simulink model "ZF02HD250606_23a"  (R2023a)
settings: Solver=ode4  StartTime=0.0  StopTime=inf  FixedStep=0.002  RelTol=1e-3
InitFcn:
  |  T_c = 0.002;
undefined symbols (not defined in the file): DiscIntNeverNeededParam, Discrete, magnitude, Time
libraries: AFCToolbox x33, simulink x28, simulink_extras x7, sharedtransform x2, ctrlSharedLib x2, aerolibconvert2 x1, aerolibtransform2 x1, dspstat3 x1, dspsolvers x1
(part 1 of 3)
settings Model: Creator=zqinghua  LastModifiedBy=zqhkd
settings OptimizationCC: DefaultParameterBehavior=Inlined  OptimizeBlockIOStorage=off  BufferReuse=off  ReuseModelBlockBuffer=off  GlobalBufferReuse=off  ExpressionFolding=off  EnableMemcpy=off  PassReuseOutputArgsAs=Individual arguments  LocalBlockOutputs=off  ZeroExternalMemoryAtStartup=off  ZeroInternalMemoryAtStartup=off  OptimizeDataStoreBuffers=off  BusAssignmentInplaceUpdate=off  OptimizationLevel=level0  OptimizationCustomize=off  EfficientTunableParamExpr=on
settings DebuggingCC: ParameterOverflowMsg=none  ParameterUnderflowMsg=error  ParameterTunabilityLossMsg=error
settings HardwareCC: ProdBitPerInt=16  ProdBitPerPointer=16  ProdBitPerSizeT=16  ProdBitPerPtrDiffT=16  ProdLargestAtomicFloat=None  ProdWordSize=16  ProdHWDeviceType=STMicroelectronics->ST10/Super10  TargetBitPerInt=16  TargetBitPerPointer=16  TargetBitPerSizeT=16  TargetBitPerPtrDiffT=16  TargetIntDivRoundTo=Zero  TargetEndianess=LittleEndian  TargetWordSize=16  TargetHWDeviceType=STMicroelectronics->ST10/Super10
settings SFSimCC: MATLABDynamicMemAlloc=off
settings RTWCC: Description=Embedded Coder  SystemTargetFile=AFCHawk.tlc  GenCodeOnly=on  TemplateMakefile=ert_default_tmf
settings CodeAppCC: ForceParamTrailComments=on  IgnoreCustomStorageClasses=off  OperatorAnnotations=on  SimulinkDataObjDesc=on  SFDataObjDesc=on  InsertBlockDesc=on
settings STFCustomTargetCC: MultiwordLength=256  ModelReferenceCompliant=off  ConcurrentExecutionCompliant=off  CombineOutputUpdateFcns=on  ERTCustomFileBanners=on  SupportContinuousTime=off  SupportNonInlinedSFcns=off  RemoveResetFunc=on  MATLABClassNameForMDSCustomization=Simulink.SoftwareTarget.ERTCustomization  GRTInterface=off  UseToolchainInfoCompliant=off  SystemTargetFile=AFCHawk.tlc
settings ERTTargetCC: TargetLangStandard=C99 (ISO)  ModelReferenceCompliant=off  ParMdlRefBuildCompliant=off  CompOptLevelCompliant=off  ConcurrentExecutionCompliant=off  ModelStepFunctionPrototypeControlCompliant=off  CPPClassGenCompliant=off  UseToolchainInfoCompliant=off  InlinedParameterPlacement=NonHierarchical  ERTCustomFileTemplate=example_file_process.tlc
settings ConfigComp: CovBoundaryAbsTol=1.0e-5

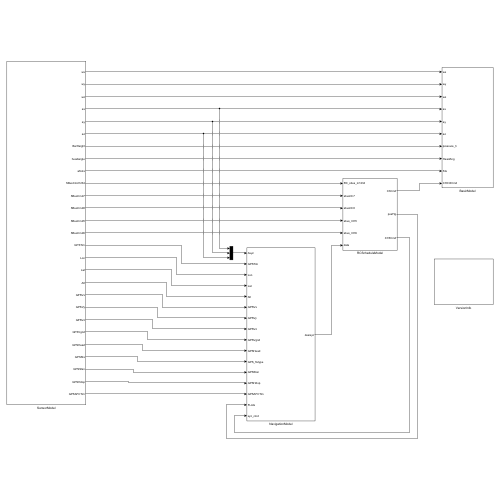
[thumbnail: Simulink's stored preview of the top-level diagram]
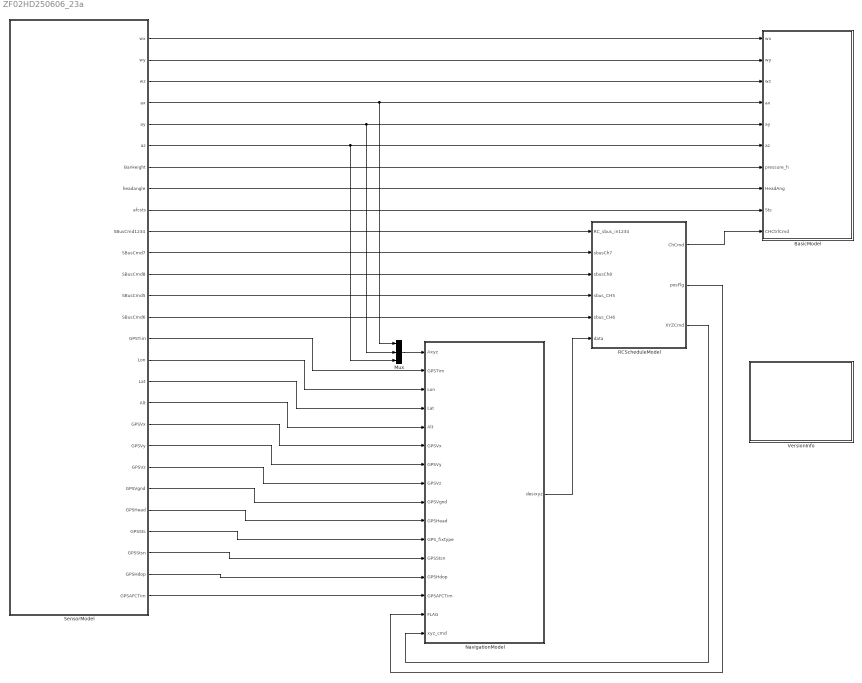
== system ZF02HD250606_23a ==
  BasicModel : Subsystem
  Mux : Mux  Inputs=3
  NavigationModel : Subsystem
  RCScheduleModel : Subsystem
  SensorModel : Subsystem
  VersionInfo : Subsystem
  wires:
  RCScheduleModel/1(ChCmd) -> BasicModel/10(CHCtrlCmd)
  SensorModel/8(headangle) -> BasicModel/8(HeadAng)
  SensorModel/21(GPSVz) -> NavigationModel/8(GPSVz)
  SensorModel/20(GPSVy) -> NavigationModel/7(GPSVy)
  SensorModel/23(GPSHead) -> NavigationModel/10(GPSHead)
  SensorModel/4(ax) -> Mux/1, BasicModel/4(ax)
  SensorModel/18(Alt) -> NavigationModel/5(Alt)
  SensorModel/25(GPSStsn) -> NavigationModel/12(GPSStsn)
  SensorModel/17(Lat) -> NavigationModel/4(Lat)
  SensorModel/19(GPSVx) -> NavigationModel/6(GPSVx)
  SensorModel/7(BarHeight) -> BasicModel/7(pressure_h)
  RCScheduleModel/3(XYZCmd) -> NavigationModel/16(xyz_cmd)
  NavigationModel/1(desixyz) -> RCScheduleModel/6(data)
  SensorModel/27(GPSAFCTim) -> NavigationModel/14(GPSAFCTim)
  SensorModel/16(Lon) -> NavigationModel/3(Lon)
  SensorModel/24(GPSSts) -> NavigationModel/11(GPS_fixtype)
  RCScheduleModel/2(posFlg) -> NavigationModel/15(FLAG)
  SensorModel/9(afcsts) -> BasicModel/9(Sts)
  SensorModel/15(GPSTim) -> NavigationModel/2(GPSTim)
  SensorModel/1(wx) -> BasicModel/1(wx)
  SensorModel/26(GPSHdop) -> NavigationModel/13(GPSHdop)
  SensorModel/12(SBusCmd8) -> RCScheduleModel/3(sbusCh8)
  SensorModel/11(SBusCmd7) -> RCScheduleModel/2(sbusCh7)
  SensorModel/14(SBusCmd6) -> RCScheduleModel/5(sbus_CH6)
  SensorModel/22(GPSVgnd) -> NavigationModel/9(GPSVgnd)
  SensorModel/10(SBusCmd1234) -> RCScheduleModel/1(RC_sbus_in1234)
  SensorModel/6(az) -> Mux/3, BasicModel/6(az)
  SensorModel/3(wz) -> BasicModel/3(wz)
  SensorModel/13(SBusCmd5) -> RCScheduleModel/4(sbus_CH5)
  SensorModel/2(wy) -> BasicModel/2(wy)
  SensorModel/5(ay) -> Mux/2, BasicModel/5(ay)
  Mux/1 -> NavigationModel/1(Axyz)

== system ZF02HD250606_23a/BasicModel ==
  note: 起飞前检查数据
  note: 飞行分析用的详细监测数据
  wx : Inport
  wy : Inport  Port=2
  wz : Inport  Port=3
  ax : Inport  Port=4
  ay : Inport  Port=5
  az : Inport  Port=6
  pressure_h : Inport  Port=7
  HeadAng : Inport  Port=8
  Sts : Inport  Port=9
  CHCtrlCmd : Inport  Port=10
  AttiAltHold : Subsystem
  Data Type Conversion : DataTypeConversion  OutDataTypeStr=double  SaturateOnIntegerOverflow=off  RndMeth=Floor
  Tx02 : Subsystem
  Tx03 : Subsystem
  ZF02无人机 : Subsystem  Priority=6
  tag scope: flySts=global, pwm=global
  wires:
  pressure_h/1 -> AttiAltHold/7(pressure_h)
  wz/1 -> AttiAltHold/3(Wz)
  wy/1 -> AttiAltHold/2(Wy)
  wx/1 -> AttiAltHold/1(Wx)
  ax/1 -> AttiAltHold/4(Ax)
  az/1 -> AttiAltHold/6(Az)
  ay/1 -> AttiAltHold/5(Ay)
  CHCtrlCmd/1 -> AttiAltHold/10(CHCtrlCmd)
  HeadAng/1 -> AttiAltHold/8(HeadAng)
  Sts/1 -> AttiAltHold/9(Sts)
  AttiAltHold/1(MotorOut) -> ZF02无人机/1(MotorVal), [pwm]
  AttiAltHold/2(flySts) -> ZF02无人机/2(FlySts), Data Type Conversion/1
  Data Type Conversion/1 -> [flySts]

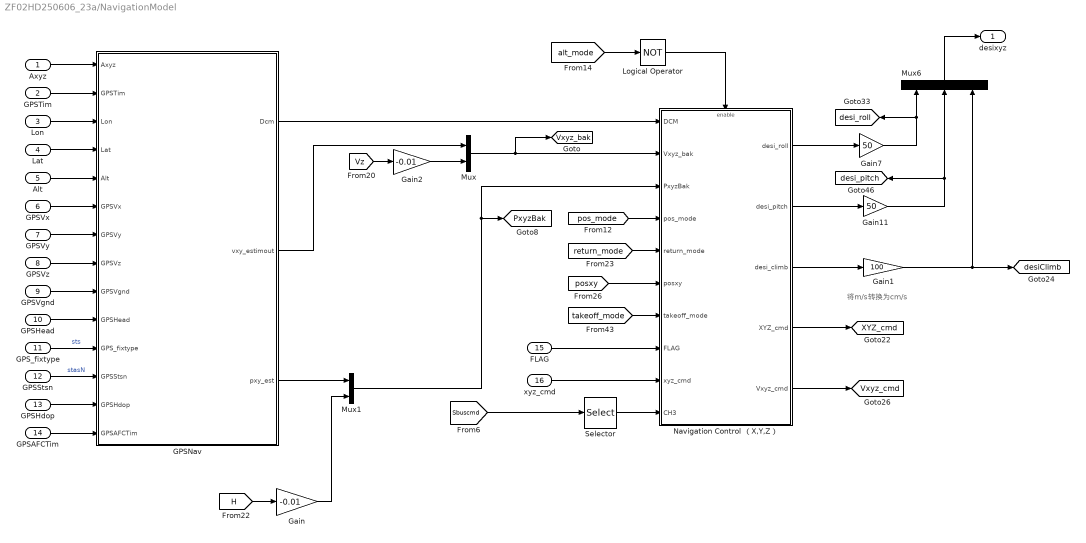
== system ZF02HD250606_23a/NavigationModel ==
  note: 将m/s转换为cm/s
  Axyz : Inport
  GPSTim : Inport  Port=2
  Lon : Inport  Port=3
  Lat : Inport  Port=4
  Alt : Inport  Port=5
  GPSVx : Inport  Port=6
  GPSVy : Inport  Port=7
  GPSVz : Inport  Port=8
  GPSVgnd : Inport  Port=9
  GPSHead : Inport  Port=10
  GPS_fixtype : Inport  Port=11
  GPSStsn : Inport  Port=12
  GPSHdop : Inport  Port=13
  GPSAFCTim : Inport  Port=14
  FLAG : Inport  Port=15
  xyz_cmd : Inport  Port=16
  " Navigation Control （X,Y,Z）" : Subsystem
  GPSNav : Subsystem
  Gain : Gain  Gain=-0.01
  Gain1 : Gain  Gain=100
  Gain11 : Gain  Gain=50
  Gain2 : Gain  Gain=-0.01
  Gain7 : Gain  Gain=50
  Logical Operator : Logic  Operator=NOT  AllPortsSameDT=off  OutDataTypeStr=boolean
  Mux : Mux  Inputs=2
  Mux1 : Mux  Inputs=2
  Mux6 : Mux  Inputs=3
  Selector : Selector  InputPortWidth=4  IndexOptions=Index vector (dialog)  Indices=3  OutputSizes=1
  desixyz : Outport
  tag scope: PxyzBak=global, Vxyz_bak=global, Vxyz_cmd=global, XYZ_cmd=global, desiClimb=global, desi_pitch=global, desi_roll=global
  wires:
  xyz_cmd/1 -> " Navigation Control （X,Y,Z）"/9(xyz_cmd)
  Mux6/1 -> desixyz/1
  FLAG/1 -> " Navigation Control （X,Y,Z）"/8(FLAG)
  Gain1/1 -> Mux6/3, [desiClimb]
  [H] -> Gain/1
  [takeoff_mode] -> " Navigation Control （X,Y,Z）"/7(takeoff_mode)
  " Navigation Control （X,Y,Z）"/3(desi_climb) -> Gain1/1
  [pos_mode] -> " Navigation Control （X,Y,Z）"/4(pos_mode)
  Logical Operator/1 -> " Navigation Control （X,Y,Z）"/Enable
  [return_mode] -> " Navigation Control （X,Y,Z）"/5(return_mode)
  [posxy] -> " Navigation Control （X,Y,Z）"/6(posxy)
  " Navigation Control （X,Y,Z）"/1(desi_roll) -> Gain7/1
  " Navigation Control （X,Y,Z）"/2(desi_pitch) -> Gain11/1
  " Navigation Control （X,Y,Z）"/4(XYZ_cmd) -> [XYZ_cmd]
  " Navigation Control （X,Y,Z）"/5(Vxyz_cmd) -> [Vxyz_cmd]
  Gain7/1 -> Mux6/1, [desi_roll]
  Gain11/1 -> Mux6/2, [desi_pitch]
  GPSTim/1 -> GPSNav/2(GPSTim)
  Lon/1 -> GPSNav/3(Lon)
  Lat/1 -> GPSNav/4(Lat)
  Alt/1 -> GPSNav/5(Alt)
  GPSVx/1 -> GPSNav/6(GPSVx)
  GPSVy/1 -> GPSNav/7(GPSVy)
  GPSVz/1 -> GPSNav/8(GPSVz)
  GPSVgnd/1 -> GPSNav/9(GPSVgnd)
  GPSHead/1 -> GPSNav/10(GPSHead)
  GPS_fixtype/1 -> GPSNav/11(GPS_fixtype)  "sts"
  GPSStsn/1 -> GPSNav/12(GPSStsn)  "stasN"
  GPSHdop/1 -> GPSNav/13(GPSHdop)
  GPSAFCTim/1 -> GPSNav/14(GPSAFCTim)
  [alt_mode] -> Logical Operator/1
  GPSNav/1(Dcm) -> " Navigation Control （X,Y,Z）"/1(DCM)
  GPSNav/2(vxy_estimout) -> Mux/1
  Axyz/1 -> GPSNav/1(Axyz)
  [Sbuscmd] -> Selector/1
  Selector/1 -> " Navigation Control （X,Y,Z）"/10(CH3)
  Mux/1 -> [Vxyz_bak], " Navigation Control （X,Y,Z）"/2(Vxyz_bak)
  [Vz] -> Gain2/1
  Gain2/1 -> Mux/2
  GPSNav/3(pxy_est) -> Mux1/1
  Gain/1 -> Mux1/2
  Mux1/1 -> " Navigation Control （X,Y,Z）"/3(PxyzBak), [PxyzBak]

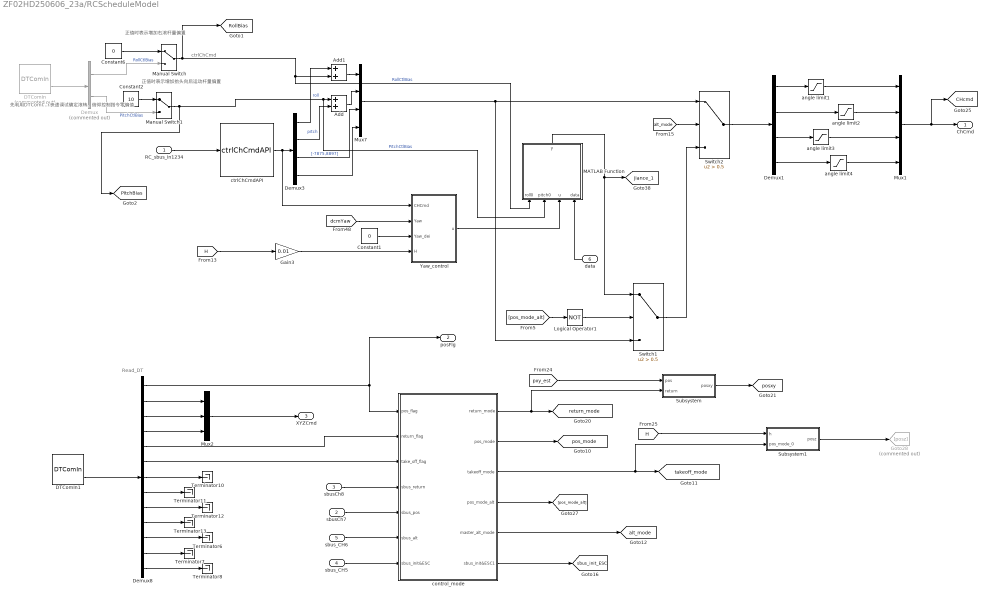
== system ZF02HD250606_23a/RCScheduleModel ==
  note: 先利用DTComIn快速调试确定滚转、俯仰控制指令零偏值
  note: 正值时表示增加右滚杆量偏置
  note: ctrlChCmd
  note: Read_DT
  note: 正值时表示增加抬头向后运动杆量偏置
  RC_sbus_in1234 : Inport
  sbusCh7 : Inport  Port=2
  sbusCh8 : Inport  Port=3
  sbus_CH5 : Inport  Port=4
  sbus_CH6 : Inport  Port=5
  data : Inport  Port=6
  Add : Sum
  Add1 : Sum
  Constant1 : Constant  Value=0
  Constant2 : Constant  Value=10
  Constant6 : Constant  Value=0
  DTComIn : AFCToolbox/DeviceModule/DTComIn  Priority=2  Commented=on  g_sampleTime=0.01  g_frameType=22  g_resFrameNum=0  g_comPort=6  g_instName=0  g_id=0
      settings: SourceProductName=AFCToolbox
  DTComIn1 : AFCToolbox/DeviceModule/DTComIn  Priority=2  g_sampleTime=0.01  g_frameType=25  g_resFrameNum=0  g_comPort=6  g_instName=0  g_id=0
      settings: SourceProductName=AFCToolbox
  Demux : Demux  Commented=on  Outputs=2
  Demux1 : Demux
  Demux3 : Demux
  Demux8 : Demux  Outputs=13
  Gain3 : Gain  Gain=0.01
  Goto28 : Goto  Commented=on  GotoTag=posz
  Logical Operator1 : Logic  Operator=NOT  AllPortsSameDT=off  OutDataTypeStr=boolean
  MATLAB Function : MATLAB Function  TreatAsAtomicUnit=on
  Manual Switch : ManualSwitch
  Manual Switch1 : ManualSwitch
  Mux1 : Mux
  Mux2 : Mux  Inputs=3
  Mux7 : Mux
  Subsystem : Subsystem
  Subsystem1 : Subsystem
  Switch1 : Switch  Criteria=u2 > Threshold  Threshold=0.5  SaturateOnIntegerOverflow=off  InputSameDT=off
  Switch2 : Switch  Criteria=u2 > Threshold  Threshold=0.5  SaturateOnIntegerOverflow=off  InputSameDT=off
  Terminator{6..8,10..13} (7 alike) : Terminator
  Yaw_control : Subsystem
  angle limit1 : Saturate  UpperLimit=1500  LowerLimit=-1500
  angle limit2 : Saturate  UpperLimit=1500  LowerLimit=-1500
  angle limit3 : Saturate  UpperLimit=10500  LowerLimit=-10500
  angle limit4 : Saturate  UpperLimit=250  LowerLimit=-250
  control_mode : Subsystem
  ctrlChCmdAPI : AFCToolbox/APPModule/ctrlChCmdAPI  Priority=3
      settings: SourceProductName=AFCToolbox
  ChCmd : Outport
  posFlg : Outport  Port=2
  XYZCmd : Outport  Port=3
  tag scope: CHcmd=global, PitchBias=global, RollBias=global, alt_mode=global, jiance_1=global, pos_mode=global, posxy=global, return_mode=global, sbus_init_ESC=global, takeoff_mode=global
  wires:
  Demux3/4 -> Mux7/4
  [pxy_est] -> Subsystem/1(pos)
  [pos_mode_alt] -> Logical Operator1/1
  ctrlChCmdAPI/1 -> Demux3/1, Yaw_control/1(CHCmd)
  Switch1/1 -> Switch2/3
  Manual Switch/1 -> [RollBias], Add1/2, MATLAB Function/1(roll0)  "RollCtlBias"
  Manual Switch1/1 -> [PitchBias], MATLAB Function/2(pitch0), Add/1  "PitchCtlBias"
  Add1/1 -> Mux7/1
  Demux3/1 -> Add1/1  "roll"
  Demux8/11 -> Terminator6/1
  Demux8/1 -> posFlg/1, control_mode/1(pos_flag)
  Demux3/2 -> Add/2  "pitch"
  Demux3/3 -> Mux7/3  "[-7875,8897]"
  Add/1 -> Mux7/2
  Mux7/1 -> Switch1/3, Switch2/1
  Demux8/3 -> Mux2/2
  Demux8/2 -> Mux2/1
  Demux8/4 -> Mux2/3
  [alt_mode] -> Switch2/2
  Demux8/7 -> Terminator10/1
  [H] -> Subsystem1/1(h)
  Demux8/8 -> Terminator11/1
  Demux8/9 -> Terminator12/1
  sbusCh8/1 -> control_mode/4(sbus_return)
  Demux8/10 -> Terminator13/1
  Yaw_control/1(u) -> MATLAB Function/3(u)
  Demux8/12 -> Terminator7/1
  Demux8/13 -> Terminator8/1
  control_mode/4(pos_mode_alt) -> [pos_mode_alt]
  RC_sbus_in1234/1 -> ctrlChCmdAPI/1
  control_mode/3(takeoff_mode) -> [takeoff_mode], Subsystem1/2(pos_mode_0)
  [H] -> Gain3/1
  sbusCh7/1 -> control_mode/5(sbus_pos)
  [dcmYaw] -> Yaw_control/2(Yaw)
  Constant1/1 -> Yaw_control/3(Yaw_dei)
  Gain3/1 -> Yaw_control/4(H)
  sbus_CH6/1 -> control_mode/6(sbus_alt)
  sbus_CH5/1 -> control_mode/7(sbus_init&ESC)
  control_mode/1(return_mode) -> Subsystem/2(return), [return_mode]
  control_mode/2(pos_mode) -> [pos_mode]
  control_mode/5(master_alt_mode) -> [alt_mode]
  control_mode/6(sbus_init&ESC1) -> [sbus_init_ESC]
  MATLAB Function/1(y) -> Switch1/1, [jiance_1]
  Logical Operator1/1 -> Switch1/2
  Subsystem1/1(posz) -> Goto28/1
  Subsystem/1(posxy) -> [posxy]
  data/1 -> MATLAB Function/4(data)
  Demux8/6 -> control_mode/3(take_off_flag)
  Demux8/5 -> control_mode/2(return_flag)
  Mux2/1 -> XYZCmd/1
  DTComIn1/2 -> Demux8/1
  angle limit3/1 -> Mux1/3
  angle limit4/1 -> Mux1/4
  Demux1/4 -> angle limit4/1
  angle limit1/1 -> Mux1/1
  Switch2/1 -> Demux1/1
  angle limit2/1 -> Mux1/2
  Demux1/2 -> angle limit2/1
  Mux1/1 -> [CHcmd], ChCmd/1
  Demux1/3 -> angle limit3/1
  Demux1/1 -> angle limit1/1
  DTComIn/2 -> Demux/1
  Demux/1 -> Manual Switch/2  "RollCtlBias"
  Constant6/1 -> Manual Switch/1
  Demux/2 -> Manual Switch1/2  "PitchCtlBias"
  Constant2/1 -> Manual Switch1/1

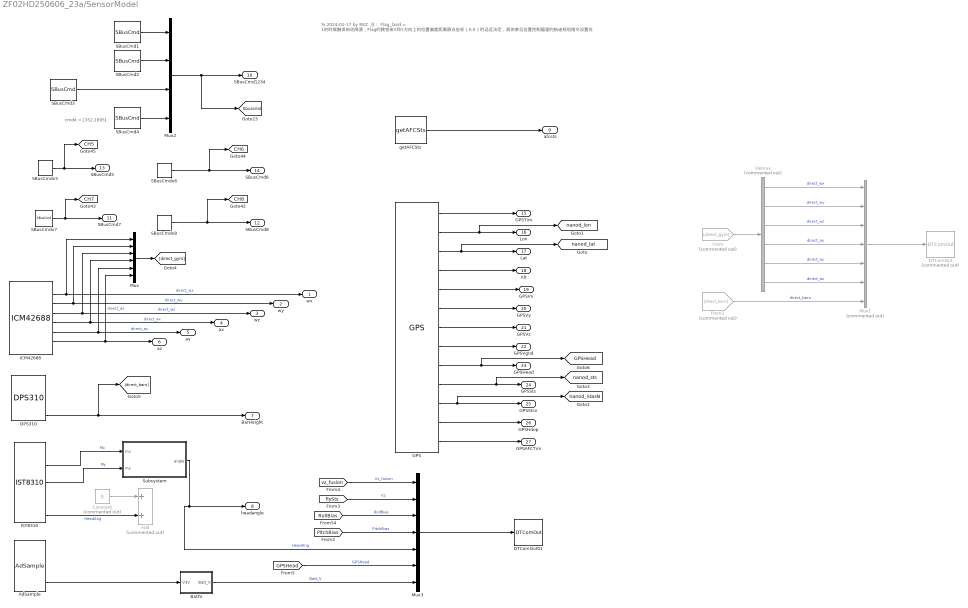
== system ZF02HD250606_23a/SensorModel ==
  note: % 2024-01-17 by REZ
      | 注：
      | Flag_land = 1的时候触发自动降落，Flag的跳变由X和Y方向上的位置偏差距离原点坐标（0,0）的远近决定，具体参见位置控制器里的航迹规划指令设置处
  note: cmd4 = [352,1695]
  AdSample : AFCToolbox/DeviceModule/AdSample  Priority=1  g_sampleTime=0.01  g_comPort=0  g_instName=0  g_id=0
      settings: SourceProductName=AFCToolbox
  Add : Sum  Commented=on
  BattV : Subsystem
  Constant : Constant  Commented=on  Value=0
  DPS310 : AFCToolbox/DeviceModule/DPS310  Priority=1  g_sampleTime=0.01  g_comPort=6  g_instName=0  g_id=0
      settings: SourceProductName=AFCToolbox
  DTComOut : AFCToolbox/DeviceModule/DTComOut  Priority=8  Commented=on  g_frameType=4  g_outFreq=10  g_comPort=0  g_instName=0  g_id=0
      settings: SourceProductName=AFCToolbox
  DTComOut01 : AFCToolbox/DeviceModule/DTComOut  Priority=8  g_frameType=1  g_outFreq=30  g_comPort=0  g_instName=0  g_id=0
      settings: SourceProductName=AFCToolbox
  Demux : Demux  Commented=on  Outputs=6
  From : From  Commented=on  GotoTag=direct_gyro
  From1 : From  Commented=on  GotoTag=direct_baro
  GPS : AFCToolbox/DeviceModule/GPS  Priority=1  g_sampleTime=T_c  g_gpsDev=M10 GNSS  g_comPort=6  g_instName=0  g_id=0
      settings: SourceProductName=AFCToolbox
  ICM42688 : AFCToolbox/DeviceModule/ICM42688  Priority=0  g_sampleTime=T_c  g_comPort=6  g_instName=0  g_id=0
      settings: SourceProductName=AFCToolbox
  IST8310 : AFCToolbox/DeviceModule/IST8310  Priority=1  g_sampleTime=0.01  g_comPort=0  g_instName=0  g_id=0
      settings: SourceProductName=AFCToolbox
  Mux : Mux  Inputs=6
  Mux1 : Mux  Commented=on  Inputs=7
  Mux2 : Mux
  Mux3 : Mux  Inputs=7
  SBusCmd1 : AFCToolbox/DeviceModule/SBusCmd  Priority=0  g_sampleTime=T_c  g_chanelNo=1  g_comPort=6  g_instName=0  g_id=0
      settings: SourceProductName=AFCToolbox
  SBusCmd2 : AFCToolbox/DeviceModule/SBusCmd  Priority=0  g_sampleTime=T_c  g_chanelNo=2  g_comPort=6  g_instName=0  g_id=0
      settings: SourceProductName=AFCToolbox
  SBusCmd3 : AFCToolbox/DeviceModule/SBusCmd  Priority=0  g_sampleTime=T_c  g_chanelNo=3  g_comPort=6  g_instName=0  g_id=0
      settings: SourceProductName=AFCToolbox
  SBusCmd4 : AFCToolbox/DeviceModule/SBusCmd  Priority=0  g_sampleTime=T_c  g_chanelNo=4  g_comPort=6  g_instName=0  g_id=0
      settings: SourceProductName=AFCToolbox
  SBusCmdx5 : AFCToolbox/DeviceModule/SBusCmd  Priority=0  g_sampleTime=T_c  g_chanelNo=5  g_comPort=6  g_instName=0  g_id=0
      settings: SourceProductName=AFCToolbox
  SBusCmdx6 : AFCToolbox/DeviceModule/SBusCmd  Priority=0  g_sampleTime=T_c  g_chanelNo=6  g_comPort=6  g_instName=0  g_id=0
      settings: SourceProductName=AFCToolbox
  SBusCmdx7 : AFCToolbox/DeviceModule/SBusCmd  Priority=0  g_sampleTime=0.002  g_chanelNo=7  g_comPort=6  g_instName=0  g_id=0
      settings: SourceProductName=AFCToolbox
  SBusCmdx8 : AFCToolbox/DeviceModule/SBusCmd  Priority=0  g_sampleTime=T_c  g_chanelNo=8  g_comPort=6  g_instName=0  g_id=0
      settings: SourceProductName=AFCToolbox
  Subsystem : Subsystem
  getAFCSts : AFCToolbox/APPModule/getAFCSts  Priority=0  g_sampleTime=T_c
      settings: SourceProductName=AFCToolbox
  wx : Outport
  wy : Outport  Port=2
  wz : Outport  Port=3
  ax : Outport  Port=4
  ay : Outport  Port=5
  az : Outport  Port=6
  BarHeight : Outport  Port=7
  headangle : Outport  Port=8
  afcsts : Outport  Port=9
  SBusCmd1234 : Outport  Port=10
  SBusCmd7 : Outport  Port=11
  SBusCmd8 : Outport  Port=12
  SBusCmd5 : Outport  Port=13
  SBusCmd6 : Outport  Port=14
  GPSTim : Outport  Port=15
  Lon : Outport  Port=16
  Lat : Outport  Port=17
  Alt : Outport  Port=18
  GPSVx : Outport  Port=19
  GPSVy : Outport  Port=20
  GPSVz : Outport  Port=21
  GPSVgnd : Outport  Port=22
  GPSHead : Outport  Port=23
  GPSSts : Outport  Port=24
  GPSStsn : Outport  Port=25
  GPSHdop : Outport  Port=26
  GPSAFCTim : Outport  Port=27
  tag scope: CH5=global, CH6=global, CH7=global, CH8=global, GPSHead=global, Sbuscmd=global, nanod_StasN=global, nanod_lat=global, nanod_lon=global, nanod_sts=global
  wires:
  GPS/1 -> GPSTim/1
  GPS/2 -> [nanod_lon], Lon/1
  GPS/3 -> [nanod_lat], Lat/1
  GPS/4 -> Alt/1
  SBusCmd1/1 -> Mux2/1
  SBusCmd2/1 -> Mux2/2
  SBusCmd3/1 -> Mux2/3
  SBusCmd4/1 -> Mux2/4
  SBusCmdx7/1 -> [CH7], SBusCmd7/1
  getAFCSts/1 -> afcsts/1
  SBusCmdx8/1 -> [CH8], SBusCmd8/1
  SBusCmdx6/1 -> [CH6], SBusCmd6/1
  GPS/12 -> GPSHdop/1
  DPS310/4 -> [direct_baro], BarHeight/1
  GPS/11 -> GPSStsn/1, [nanod_StasN]
  ICM42688/2 -> Mux/1, wx/1  "direct_wx"
  ICM42688/5 -> Mux/4, ax/1  "direct_ax"
  GPS/7 -> GPSVz/1
  GPS/8 -> GPSVgnd/1
  SBusCmdx5/1 -> [CH5], SBusCmd5/1
  GPS/5 -> GPSVx/1
  GPS/6 -> GPSVy/1
  GPS/9 -> [GPSHead], GPSHead/1
  GPS/10 -> [nanod_sts], GPSSts/1
  GPS/13 -> GPSAFCTim/1
  Mux2/1 -> [Sbuscmd], SBusCmd1234/1
  ICM42688/3 -> Mux/2, wy/1  "direct_wy"
  ICM42688/6 -> Mux/5, ay/1  "direct_ay"
  ICM42688/4 -> Mux/3, wz/1  "direct_wz"
  ICM42688/7 -> Mux/6, az/1  "direct_az"
  Mux/1 -> [direct_gyro]
  From1/1 -> Mux1/7  "direct_baro"
  Demux/6 -> Mux1/6  "direct_az"
  Mux1/1 -> DTComOut/1
  Demux/1 -> Mux1/1  "direct_wx"
  Demux/2 -> Mux1/2  "direct_wy"
  Demux/4 -> Mux1/4  "direct_ax"
  Demux/3 -> Mux1/3  "direct_wz"
  Demux/5 -> Mux1/5  "direct_ay"
  From/1 -> Demux/1
  Subsystem/1(angle) -> Mux3/5, headangle/1  "HeadAng"
  AdSample/3 -> BattV/1(V3V)
  Mux3/1 -> DTComOut01/1
  [RollBias] -> Mux3/3  "RollBias"
  [flySts] -> Mux3/2  "Vz"
  [vz_fusion] -> Mux3/1  "Vz_fusion"
  [PitchBias] -> Mux3/4  "PitchBias"
  BattV/1(Batt_V) -> Mux3/7  "Batt_V"
  IST8310/5 -> Add/2  "HeadAng"
  Constant/1 -> Add/1
  [GPSHead] -> Mux3/6  "GPSHead"
  IST8310/3 -> Subsystem/2(my)  "My"
  IST8310/2 -> Subsystem/1(mx)  "Mx"

== system ZF02HD250606_23a/VersionInfo ==
  note: % 2024-01-11 Positon Controller 修改 ， by REZ
      |
      | 1.积分器重置条件，根据油门，已知实际遥控器CH3>0.4左右开始离地，离地前需要进行积分器重置； 遥控器的CH3=0.3-0.4左右对应在模型中Cmd_ch3=880，即重置条件为：当Ch3<880进行积分重置。
      |
      | 2.积分器的限幅范围：对位置控制器里的四个积分器暂时施加了[-3,3]的限幅，主要考虑当x和y方向的位置误差最大在3m内的时候，单纯由积分器得到的控制量不能占据PID控制器主导量而导致控制异常！
      |
      | %2024-01-15:
      | 位置控制器重修，P-PID控制器参数修改了一版；积分限幅
      |
      | % 2024-01-16：
      | 修改增加了一个含逻辑切换的正方形航迹规划指令；
      |
      | %2024-01-19:
      | 航迹规划的优化及飞行验证；
      |
      | %22024-03-08：
      | 增加control_mode模式选择模块：
      | （1）ch5为sbus_init_ESC开关同时进行电调控制解锁与导航初始化，其不受其他模式影响；
      | （2）ch6为高度控制与位置模式的切换通道，通道置1为高度控制模式，否则将进行位置控制模式，在所有模式中高度控制模式优先级最高，只要该通道置1，其他模式将不起作用；
      | （3）ch7为位置控制模式，该模式优先级最低，主要进行航迹飞行，其他通道置零，ch7通道置1，进行预设点飞行，否则进入（0,0,h）定点模式，定点模式可以理解为航迹规划前的无人机位置调整与准备；
      | （4）ch8为返航控制模式，该模式优先级高于航迹控制，但低于高度控制模式，通道置1，无人机将进行返航任务。
      |
      | %22024-03-08：
      | 优化位置控制模块，可随意更改航迹点，并预留与上位机进行点位设置的接口模块。注意，该版本航迹飞行为平面飞行，未涉及到高度，因此在进行点位设置时，只需设计X和Y两个方向的点位，可自行在setpoints封装模块的MASK界面进行修改，同时可修改触发阈值。
      |
      | %22024-03-10：
      | 优化位置控制，同时增加返航模块。将位置控制模式划分为三个模 式，（0,0）定点模式，航迹规划模式，一键返航模式，与control_mode相对应，通过遥控器对应拨杆进行模式切换。
      | （1）三个模式共用同一组控制参数，（0,0）定点模式和航迹规划模式不进行高度控制，保持当前高度；
      | （2）一键返航模式任务要求，无人机接收到指令后，首先保持水平位置，进行高度方向的飞行，达到决断高度之后，无人机保持当前高度h0,然后向（0,0,h）点位飞行，随后无人机进行降落。
      | （3）将位置模式产生的上升率与下降率叠加到遥控器指令生成的控制率中。
      |
      | %22024-03-11：
      | 优化位置控制，可进行三维空间点位设置。
      |
      | %22024-03-12：
      | 取消pos_mode(0,0)模式，优化三维航迹，无人机接受指令后，先飞行高度，随后进行水平飞行。
      |
      | %22024-03-14：
      | 优化返航模式，解决了返航复飞的现象。
      |
      | %22024-03-14：
      | 增加了定点模式，航迹飞行前，无人机先进行当前高度的单定点飞行，验证其飞行性能，随后进行三维航迹飞行。
      |
      | %22024-03-14：
      | 加入偏航控制模式，使其一直处于正北方向。
      |
      | %22024-03-15：
      | 增加上位机点位设置模块。
      |
      | %22024-03-16：
      | 将偏航控制单独加到位置控制模式；
      |
      | %22024-03-17：
      | 增加一键起飞模式，无人机解锁，同时油门至中位，此时，将遥控器7号拨杆至中位，无人机进行一键起飞。
      |
      | %22024-03-18：
      | 简化三维航迹飞行，同时进行高度与水平飞行。
      | %22024-03-22：
      | 优化偏航控制，在飞行高度大于0.5米，偏航控制有效。
      | %22024-03-24：
      | 优化上位机控制逻辑，实现遥控控制与上位机控制相互兼容，上位机可发送起飞指令，返航指令，三维坐标点。
      | %22024-05-15:
      | F550-4 飞8m；未加磁力计补偿，yaw的kp参数需要在线调参为6.6；
      |
      | %22024-11-05:
      | HS03 飞行正常；
      |
      | %2024-11-09：
      | . 删除SensorModel中的DTComIn, 将相应功能移至RCScheduleModel模块中；
      | . 恢复HS620PN241105.slx中setpoints1、return_mode1中删除的微分跟踪器TD模块；
      | . 在control_mode模块中，对于位置、起飞/降落等模块的触发设置一个总开关与模块PosCtlSwitch，以防止T20241105_111134出现的故障；
      |
      | V5.05.241204：根据HS620PN241111(T20241112_083920飞行的V2.424版本更改)

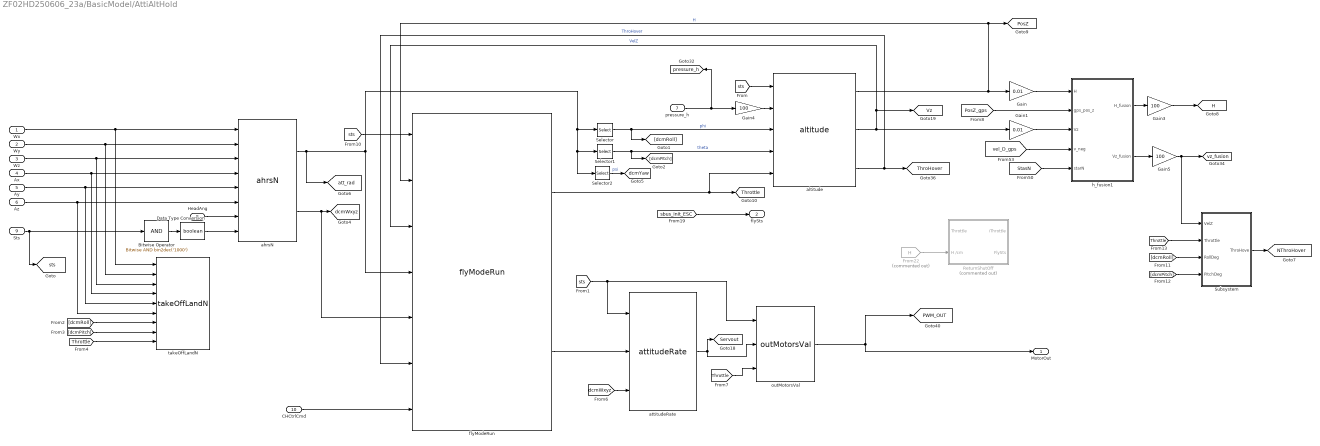
== system ZF02HD250606_23a/BasicModel/AttiAltHold ==
  Wx : Inport
  Wy : Inport  Port=2
  Wz : Inport  Port=3
  Ax : Inport  Port=4
  Ay : Inport  Port=5
  Az : Inport  Port=6
  pressure_h : Inport  Port=7
  HeadAng : Inport  Port=8
  Sts : Inport  Port=9
  CHCtrlCmd : Inport  Port=10
  Bitwise Operator : simulink/Logic and Bit Operations/Bitwise Operator  logicop=AND  UseBitMask=on  BitMask=bin2dec('1000')  BitMaskRealWorld=Stored Integer
  Data Type Conversion : DataTypeConversion  OutDataTypeStr=boolean  SaturateOnIntegerOverflow=off  RndMeth=Floor
  From22 : From  Commented=on  GotoTag=H  TagVisibility=global
  Gain : Gain  Gain=0.01
  Gain1 : Gain  Gain=0.01
  Gain3 : Gain  Gain=100
  Gain4 : Gain  Gain=100
  Gain5 : Gain  Gain=100
  ReturnShutOff : Subsystem  Commented=on
  Selector : Selector  InputPortWidth=3  IndexOptions=Index vector (dialog)  Indices=1  OutputSizes=1
  Selector1 : Selector  InputPortWidth=3  IndexOptions=Index vector (dialog)  Indices=2  OutputSizes=1
  Selector2 : Selector  InputPortWidth=3  IndexOptions=Index vector (dialog)  Indices=3  OutputSizes=1
  Subsystem : Subsystem
  ahrsN : AFCToolbox/APPModule/ahrsN  Priority=3  kp=0.14  ki=0.0087  kp_yaw=0.16  ki_yaw=0.001  dt=0.002  g=9.80665
      settings: SourceProductName=AFCToolbox
  altitude : AFCToolbox/APPModule/altitude  Priority=3  alt_pos_kp=1.8  pid_alt_rate_kp=8.0  pid_alt_rate_ki=0.1  pid_alt_rate_kd=1.0  pid_alt_rate_imax=800.0  pid_alt_accel_kp=1.36  pid_alt_accel_ki=0.1  pid_alt_accel_kd=0.08  pid_alt_accel_imax=800.0  k1=0.6  k2=0.12  k3=0.008  control_dt=0.002  g=9.80665
      settings: SourceProductName=AFCToolbox
  attitudeRate : AFCToolbox/APPModule/attitudeRate  Priority=4  angle_kp0=8.0  angle_kp1=6.6  angle_kp2=8.0  pid_rate0_kp=0.32  pid_rate0_ki=0.1  pid_rate0_kd=3.5  pid_rate1_kp=0.32  pid_rate1_ki=0.1  pid_rate1_kd=3.5  pid_rate2_kp=0.6  pid_rate2_ki=0.03  pid_rate2_kd=1.5  pid_rate0_imax=500.0  pid_rate1_imax=500.0  pid_rate2_imax=500.0  max0=5000.0  min0=-5000.0  max1=5000.0  min1=-5000.0  max2=4000.0  min2=-4000.0  control_dt=0.002
      settings: SourceProductName=AFCToolbox
  flyModeRun : AFCToolbox/APPModule/flyModeRun  Priority=4
      settings: SourceProductName=AFCToolbox
  h_fusion1 : Subsystem
  outMotorsVal : AFCToolbox/APPModule/outMotorsVal  Priority=5
      settings: SourceProductName=AFCToolbox
  takeOffLandN : AFCToolbox/APPModule/takeOffLandN  Priority=5  RC_Climb_Rate=0
      settings: SourceProductName=AFCToolbox
  MotorOut : Outport
  flySts : Outport  Port=2
  tag scope: H=global, NThroHover=global, PWM_OUT=global, PosZ=global, Servout=global, ThroHover=global, Throttle=global, Vz=global, att_rad=global, dcmWxyz=global, dcmYaw=global, pressure_h=global, sts=global, vz_fusion=global
  wires:
  Selector1/1 -> [dcmPitch], altitude/4  "theta"
  Data Type Conversion/1 -> ahrsN/8
  ahrsN/2 -> flyModeRun/5, [dcmWxyz]
  attitudeRate/1 -> outMotorsVal/2, [Servout]
  Selector/1 -> altitude/3, [dcmRoll]  "phi"
  Ax/1 -> takeOffLandN/4, ahrsN/4
  Wx/1 -> takeOffLandN/1, ahrsN/1
  [Throttle] -> takeOffLandN/9
  ahrsN/1 -> [att_rad], flyModeRun/4, Selector2/1, Selector1/1, Selector/1
  [dcmRoll] -> takeOffLandN/7
  [dcmPitch] -> takeOffLandN/8
  [sts] -> altitude/1
  [dcmWxyz] -> attitudeRate/3
  outMotorsVal/1 -> MotorOut/1, [PWM_OUT]
  Selector2/1 -> [dcmYaw]  "psi"
  flyModeRun/2 -> attitudeRate/2
  [Throttle] -> outMotorsVal/3
  [sts] -> attitudeRate/1, outMotorsVal/1
  altitude/3 -> [ThroHover], flyModeRun/6  "ThroHover"
  [sts] -> flyModeRun/1
  Gain4/1 -> altitude/2
  pressure_h/1 -> [pressure_h], Gain4/1
  CHCtrlCmd/1 -> flyModeRun/7
  HeadAng/1 -> ahrsN/7
  Sts/1 -> [sts], Bitwise Operator/1
  Bitwise Operator/1 -> Data Type Conversion/1
  Wy/1 -> takeOffLandN/2, ahrsN/2
  Wz/1 -> takeOffLandN/3, ahrsN/3
  Ay/1 -> takeOffLandN/5, ahrsN/5
  Az/1 -> takeOffLandN/6, ahrsN/6
  altitude/2 -> Gain1/1, [Vz], flyModeRun/3  "VelZ"
  altitude/1 -> [PosZ], flyModeRun/2, Gain/1  "H"
  [dcmRoll] -> Subsystem/3(RollDeg)
  [dcmPitch] -> Subsystem/4(PitchDeg)
  Gain5/1 -> Subsystem/1(VelZ), [vz_fusion]
  Subsystem/1(ThroHove) -> [NThroHover]
  [Throttle] -> Subsystem/2(Throttle)
  [PosZ_gps] -> h_fusion1/2(gps_pos_z)
  h_fusion1/1(H_fusion) -> Gain3/1
  Gain/1 -> h_fusion1/1(H)
  Gain3/1 -> [H]
  Gain1/1 -> h_fusion1/3(Vz)
  [vel_D_gps] -> h_fusion1/4(v_neg)
  [StasN] -> h_fusion1/5(starN)
  h_fusion1/2(Vz_fusion) -> Gain5/1
  [sbus_init_ESC] -> flySts/1
  From22/1 -> ReturnShutOff/2(H /cm)
  flyModeRun/1 -> altitude/5, [Throttle]

== system ZF02HD250606_23a/BasicModel/Tx02 ==
  DTComOut2 : AFCToolbox/DeviceModule/DTComOut  Priority=8  g_frameType=2  g_outFreq=10  g_comPort=0  g_instName=0  g_id=0
      settings: SourceProductName=AFCToolbox
  Demux1 : Demux
  Demux12 : Demux
  Demux6 : Demux  Outputs=3
  Mux : Mux  Inputs=26
  Radians to Degrees2 : simulink_extras/Transformations/Radians to Degrees
  Subsystem2 : Subsystem
  wires:
  [pos_N_gps] -> Mux/1  "pos_N_gps"
  Demux12/2 -> Mux/16  "CH2"
  Demux6/1 -> Mux/12  "att_deg_roll"
  [CH6] -> Mux/21  "CH6"
  [nanod_sts] -> Mux/5  "nanod_sts"
  [PosZ_gps] -> Mux/3  "PosZ_gps"
  [pos_E_gps] -> Mux/2  "pos_E_gps"
  [att_rad] -> Radians to Degrees2/1
  [CH8] -> Mux/19  "CH8"
  [Sbuscmd] -> Demux12/1
  [nanod_lon] -> Mux/9, Subsystem2/2(lon_in)  "nanod_lon"
  [pressure_h] -> Mux/4  "pressure_h"
  [nanod_lat] -> Subsystem2/1(lat_in), Mux/8  "nanod_lat"
  Subsystem2/2(lon_out) -> Mux/11  "lon_jieduan"
  Radians to Degrees2/1 -> Demux6/1
  [CH5] -> Mux/22  "CH5"
  [nanod_StasN] -> Mux/7  "nanod_StasN"
  Subsystem2/1(lat_out) -> Mux/10  "lat_jieduan"
  [CH7] -> Mux/20  "CH7"
  Demux12/3 -> Mux/17  "CH3"
  Demux6/2 -> Mux/13  "att_deg_pitch"
  Demux12/4 -> Mux/18  "CH4"
  Demux6/3 -> Mux/14  "att_deg_yaw"
  Demux12/1 -> Mux/15  "CH1"
  Mux/1 -> DTComOut2/1
  Demux1/4 -> Mux/26  "CHCmd4"
  Demux1/3 -> Mux/25  "CHCmd3"
  Demux1/2 -> Mux/24  "CHCmd2"
  Demux1/1 -> Mux/23  "CHCmd1"
  [CHcmd] -> Demux1/1
  [PosZ] -> Mux/6  "PosZ"

== system ZF02HD250606_23a/BasicModel/Tx03 ==
  DTComOut2 : AFCToolbox/DeviceModule/DTComOut  Priority=8  g_frameType=3  g_outFreq=10  g_comPort=0  g_instName=0  g_id=0
      settings: SourceProductName=AFCToolbox
  Data Type Conversion : DataTypeConversion  OutDataTypeStr=double  SaturateOnIntegerOverflow=off  RndMeth=Floor
  Demux{,1,3..4,6} (5 alike) : Demux  Outputs=3
  Demux2 : Demux
  Mux : Mux  Inputs=26
  wires:
  [dcmWxyz] -> Demux4/1
  Demux/3 -> Mux/7  "pz_bak"
  Demux/1 -> Mux/5  "px_bak"
  Demux/2 -> Mux/6  "py_bak"
  Demux1/3 -> Mux/13  "vz_bak"
  Demux1/1 -> Mux/11  "vx_bak"
  Demux1/2 -> Mux/12  "vy_bak"
  Demux4/1 -> Mux/14  "dcmWx"
  Demux4/2 -> Mux/15  "dcmWy"
  Demux4/3 -> Mux/16  "dcmWz"
  Mux/1 -> DTComOut2/1
  [PxyzBak] -> Demux/1
  [Vxyz_bak] -> Demux1/1
  [pwm] -> Demux2/1
  Demux2/4 -> Mux/4  "pwm4"
  Demux2/3 -> Mux/3  "pwm3"
  Demux2/2 -> Mux/2  "pwm2"
  Demux2/1 -> Mux/1  "pwm1"
  Demux3/1 -> Mux/8  "vx_cmd"
  Demux3/2 -> Mux/9  "vy_cmd"
  Demux3/3 -> Mux/10  "vz_cmd"
  [Vxyz_cmd] -> Demux3/1
  [Throttle] -> Mux/20  "Throttle"
  Data Type Conversion/1 -> Mux/21  "AFC5Sts"
  [sts] -> Data Type Conversion/1
  [desi_roll] -> Mux/22  "desiRoll"
  [desi_pitch] -> Mux/23  "desiPitch"
  [desiClimb] -> Mux/24  "desiH"
  [ThroHover] -> Mux/25  "HoverThrottle"
  [H] -> Mux/26  "PosZ_fusion"
  Demux6/1 -> Mux/17  "X_cmd"
  Demux6/2 -> Mux/18  "Y_cmd"
  Demux6/3 -> Mux/19  "Z_cmd"
  [XYZ_cmd] -> Demux6/1  "PitchBias"

== system ZF02HD250606_23a/BasicModel/ZF02无人机 ==
  MotorVal : Inport
  FlySts : Inport  Port=2
  Constant : Constant  Value=0  OutDataTypeStr=double
  Demux1 : Demux
  HiEscCmd : AFCToolbox/DeviceModule/HiEscCmd  Priority=6  g_chanelNo=4  g_minPW=40  g_maxPW=80  g_comPort=6  g_instName=0  g_id=0
      settings: SourceProductName=AFCToolbox
  HiEscCmd1 : AFCToolbox/DeviceModule/HiEscCmd  Priority=6  g_chanelNo=5  g_minPW=40  g_maxPW=80  g_comPort=6  g_instName=0  g_id=0
      settings: SourceProductName=AFCToolbox
  HiEscCmd2 : AFCToolbox/DeviceModule/HiEscCmd  Priority=6  g_chanelNo=6  g_minPW=40  g_maxPW=80  g_comPort=6  g_instName=0  g_id=0
      settings: SourceProductName=AFCToolbox
  HiEscCmd3 : AFCToolbox/DeviceModule/HiEscCmd  Priority=6  g_chanelNo=3  g_minPW=40  g_maxPW=80  g_comPort=6  g_instName=0  g_id=0
      settings: SourceProductName=AFCToolbox
  Mux : Mux
  Switch1 : Switch  Criteria=u2 > Threshold  Threshold=0.5  SaturateOnIntegerOverflow=off  InputSameDT=off
  wires:
  MotorVal/1 -> Switch1/1
  FlySts/1 -> Switch1/2
  Switch1/1 -> Demux1/1
  Mux/1 -> Switch1/3
  Constant/1 -> Mux/4, Mux/3, Mux/2, Mux/1
  Demux1/1 -> HiEscCmd/1  "pwm1"
  Demux1/2 -> HiEscCmd1/1  "pwm2"
  Demux1/3 -> HiEscCmd2/1  "pwm3"
  Demux1/4 -> HiEscCmd3/1  "pwm4"

== system ZF02HD250606_23a/NavigationModel/ Navigation Control （X,Y,Z） ==
  DCM : Inport
  Vxyz_bak : Inport  Port=2
  PxyzBak : Inport  Port=3
  pos_mode : Inport  Port=4
  return_mode : Inport  Port=5
  posxy : Inport  Port=6
  takeoff_mode : Inport  Port=7
  FLAG : Inport  Port=8
  xyz_cmd : Inport  Port=9
  CH3 : Inport  Port=10
  Enable : EnablePort
  Compare To Constant : simulink/Logic and Bit Operations/Compare To Constant  relop=<=  const=800  OutDataTypeStr=boolean
  Logical Operator : Logic  Operator=OR  AllPortsSameDT=off  OutDataTypeStr=boolean
  POS_CONTROL : Subsystem
  SETPOINT : Subsystem
  VEL_PID : Subsystem
  desi_roll : Outport
  desi_pitch : Outport  Port=2
  desi_climb : Outport  Port=3
  XYZ_cmd : Outport  Port=4
  Vxyz_cmd : Outport  Port=5
  wires:
  VEL_PID/1(desi_roll) -> desi_roll/1
  VEL_PID/2(desi_pitch) -> desi_pitch/1
  VEL_PID/3(desi_climb) -> desi_climb/1
  return_mode/1 -> SETPOINT/3(return_mode)
  pos_mode/1 -> SETPOINT/2(pos_mode)
  SETPOINT/1(XYZ_cmd) -> XYZ_cmd/1, POS_CONTROL/1(XYZ_cmd)
  POS_CONTROL/1(Vxyz_cmd) -> Vxyz_cmd/1, VEL_PID/1(Vxyz_cmd)
  DCM/1 -> VEL_PID/2(DCM)
  Vxyz_bak/1 -> VEL_PID/3(Vxyz_bak)
  posxy/1 -> SETPOINT/1(posxy)
  takeoff_mode/1 -> SETPOINT/4(takeoff_mode)
  xyz_cmd/1 -> SETPOINT/5(xyz_cmd)
  FLAG/1 -> SETPOINT/6(FLAG)
  Logical Operator/1 -> VEL_PID/4(ClrKi), POS_CONTROL/3(ClrKi)
  CH3/1 -> Compare To Constant/1
  Compare To Constant/1 -> Logical Operator/2
  SETPOINT/2(Flag) -> Logical Operator/1
  PxyzBak/1 -> POS_CONTROL/2(XYZ_bak), SETPOINT/7(XYZ_bak)

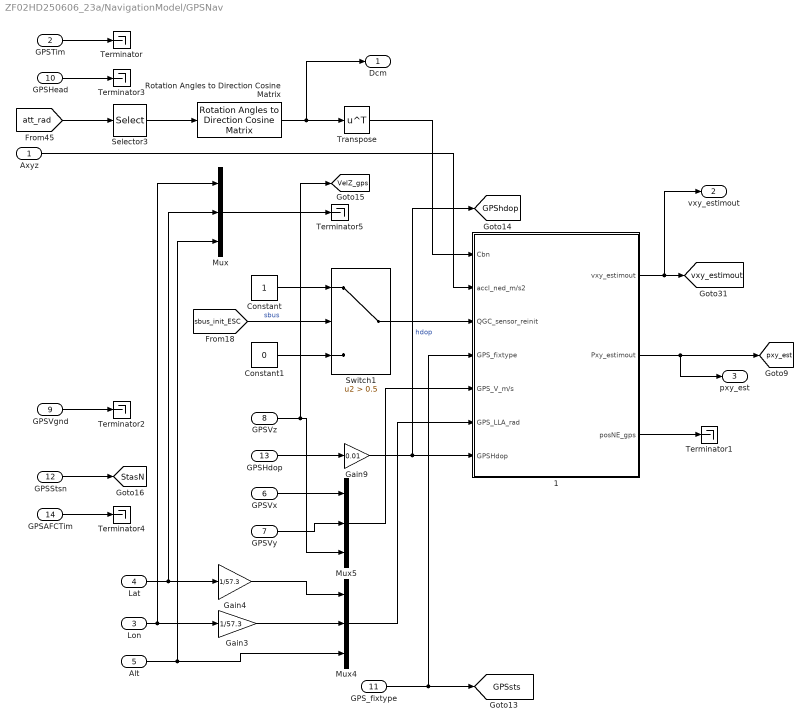
== system ZF02HD250606_23a/NavigationModel/GPSNav ==
  Axyz : Inport
  GPSTim : Inport  Port=2
  Lon : Inport  Port=3
  Lat : Inport  Port=4
  Alt : Inport  Port=5
  GPSVx : Inport  Port=6
  GPSVy : Inport  Port=7
  GPSVz : Inport  Port=8
  GPSVgnd : Inport  Port=9
  GPSHead : Inport  Port=10
  GPS_fixtype : Inport  Port=11
  GPSStsn : Inport  Port=12
  GPSHdop : Inport  Port=13
  GPSAFCTim : Inport  Port=14
  1 : Subsystem  mask{dt=0.002}
      mask prompts: dt "步长"
      mask DialogControl ParameterGroupVar Prompt: 参数
  Constant : Constant
  Constant1 : Constant  Value=0
  Gain3 : Gain  Gain=1/57.3
  Gain4 : Gain  Gain=1/57.3
  Gain9 : Gain  Gain=0.01
  Mux : Mux  Inputs=3
  Mux4 : Mux  Inputs=3
  Mux5 : Mux  Inputs=3
  Rotation Angles to Direction Cosine Matrix : sharedtransform/Rotation Angles to Direction Cosine Matrix  rotationOrder=ZYX  aMode=aMode
  Selector3 : Selector  InputPortWidth=3  IndexOptions=Index vector (dialog)  Indices=[3 2 1]  OutputSizes=1
  Switch1 : Switch  Criteria=u2 > Threshold  Threshold=0.5  SaturateOnIntegerOverflow=off  InputSameDT=off
  Terminator{,1..5} (6 alike) : Terminator
  Transpose : Math  Operator=transpose
  Dcm : Outport
  vxy_estimout : Outport  Port=2
  pxy_est : Outport  Port=3
  tag scope: GPShdop=global, GPSsts=global, StasN=global, VelZ_gps=global, pxy_est=global, vxy_estimout=global
  wires:
  GPSTim/1 -> Terminator/1
  GPSVz/1 -> [VelZ_gps], Mux5/3
  GPSStsn/1 -> [StasN]
  GPSVgnd/1 -> Terminator2/1
  GPSHead/1 -> Terminator3/1
  Gain3/1 -> Mux4/2
  Mux/1 -> Terminator5/1
  [att_rad] -> Selector3/1
  Selector3/1 -> Rotation Angles to Direction Cosine Matrix/1
  Axyz/1 -> 1/2(accl_ned_m/s2)
  GPSAFCTim/1 -> Terminator4/1
  Lat/1 -> Gain4/1, Mux/2
  GPSVy/1 -> Mux5/2
  Lon/1 -> Gain3/1, Mux/1
  Alt/1 -> Mux4/3, Mux/3
  Rotation Angles to Direction Cosine Matrix/1 -> Transpose/1, Dcm/1
  Constant1/1 -> Switch1/3
  [sbus_init_ESC] -> Switch1/2  "sbus"
  Constant/1 -> Switch1/1
  GPSHdop/1 -> Gain9/1
  GPSVx/1 -> Mux5/1
  Gain4/1 -> Mux4/1
  Transpose/1 -> 1/1(Cbn)
  Switch1/1 -> 1/3(QGC_sensor_reinit)
  Mux4/1 -> 1/6(GPS_LLA_rad)
  Gain9/1 -> 1/7(GPSHdop), [GPShdop]  "hdop"
  Mux5/1 -> 1/5(GPS_V_m/s)
  GPS_fixtype/1 -> [GPSsts], 1/4(GPS_fixtype)
  1/1(vxy_estimout) -> [vxy_estimout], vxy_estimout/1
  1/2(Pxy_estimout) -> pxy_est/1, [pxy_est]
  1/3(posNE_gps) -> Terminator1/1

== system ZF02HD250606_23a/RCScheduleModel/Subsystem ==
  pos : Inport
  return : Inport  Port=2
  Logical Operator : Logic  Operator=NOT  AllPortsSameDT=off  OutDataTypeStr=boolean
  Memory : Memory
  Switch : Switch  Criteria=u2 > Threshold  Threshold=0.5  SaturateOnIntegerOverflow=off  InputSameDT=off
  posxy : Outport
  wires:
  Switch/1 -> Memory/1, posxy/1
  Memory/1 -> Switch/3
  return/1 -> Logical Operator/1
  pos/1 -> Switch/1
  Logical Operator/1 -> Switch/2

== system ZF02HD250606_23a/RCScheduleModel/Subsystem1 ==
  h : Inport
  pos_mode_0 : Inport  Port=2
  Gain : Gain  Gain=-0.01
  Logical Operator : Logic  Operator=NOT  AllPortsSameDT=off  OutDataTypeStr=boolean
  Memory : Memory
  Switch : Switch  Criteria=u2 > Threshold  Threshold=0.5  SaturateOnIntegerOverflow=off  InputSameDT=off
  posz : Outport
  wires:
  Logical Operator/1 -> Switch/2
  h/1 -> Gain/1
  pos_mode_0/1 -> Logical Operator/1
  Memory/1 -> Switch/3
  Switch/1 -> posz/1, Memory/1
  Gain/1 -> Switch/1

== system ZF02HD250606_23a/RCScheduleModel/Yaw_control ==
  CHCmd : Inport
  Yaw : Inport  Port=2
  Yaw_dei : Inport  Port=3
  H : Inport  Port=4
  Demux9 : Demux
  MATLAB Function2 : MATLAB Function  TreatAsAtomicUnit=on
  Mux7 : Mux
  Switch : Switch  Criteria=u2 > Threshold  Threshold=0.5  SaturateOnIntegerOverflow=off  InputSameDT=off
  u : Outport
  wires:
  Demux9/1 -> Mux7/1
  Demux9/4 -> Mux7/4
  Demux9/3 -> Switch/3, MATLAB Function2/1(u)  "[-7875,8897]"
  Demux9/2 -> Mux7/2
  Mux7/1 -> u/1
  Yaw/1 -> MATLAB Function2/2(Yaw)
  CHCmd/1 -> Demux9/1
  Yaw_dei/1 -> MATLAB Function2/3(Yaw_dei)
  MATLAB Function2/1(des_wz) -> Switch/1
  H/1 -> Switch/2
  Switch/1 -> Mux7/3

== system ZF02HD250606_23a/RCScheduleModel/control_mode ==
  pos_flag : Inport
  return_flag : Inport  Port=2
  take_off_flag : Inport  Port=3
  sbus_return : Inport  Port=4
  sbus_pos : Inport  Port=5
  sbus_alt : Inport  Port=6
  sbus_init&ESC : Inport  Port=7
  Compare To Constant{,1,3..4} (4 alike) : simulink/Logic and Bit Operations/Compare To Constant  relop=>=  const=1500  OutDataTypeStr=boolean
  Compare To Constant2 : simulink/Logic and Bit Operations/Compare To Constant  relop=<  const=1500  OutDataTypeStr=boolean
  Compare To Constant5 : simulink/Logic and Bit Operations/Compare To Constant  relop=<  const=800  OutDataTypeStr=boolean
  Compare To Constant6 : simulink/Logic and Bit Operations/Compare To Constant  relop=>=  const=800  OutDataTypeStr=boolean
  Compare To Constant7 : simulink/Logic and Bit Operations/Compare To Constant  relop=>=  const=0.5  OutDataTypeStr=boolean
  Compare To Constant8 : simulink/Logic and Bit Operations/Compare To Constant  relop=>=  const=0.5  OutDataTypeStr=boolean
  Compare To Constant9 : simulink/Logic and Bit Operations/Compare To Constant  relop=>=  const=0.5  OutDataTypeStr=boolean
  Logical Operator{,3,10..11} (4 alike) : Logic  Operator=NOT  AllPortsSameDT=off  OutDataTypeStr=boolean
  Logical Operator1 : Logic  Inputs=3  AllPortsSameDT=off  OutDataTypeStr=boolean
  Logical Operator2 : Logic  Inputs=4  AllPortsSameDT=off  OutDataTypeStr=boolean
  Logical Operator4 : Logic  AllPortsSameDT=off  OutDataTypeStr=boolean
  Logical Operator5 : Logic  AllPortsSameDT=off  OutDataTypeStr=boolean
  Logical Operator6 : Logic  Inputs=5  AllPortsSameDT=off  OutDataTypeStr=boolean
  Logical Operator7 : Logic  Operator=OR  AllPortsSameDT=off  OutDataTypeStr=boolean
  Logical Operator8 : Logic  Operator=OR  AllPortsSameDT=off  OutDataTypeStr=boolean
  Logical Operator9 : Logic  Operator=OR  AllPortsSameDT=off  OutDataTypeStr=boolean
  PosCtlSwitch : Logic  AllPortsSameDT=off  OutDataTypeStr=boolean
  return_mode : Outport
  pos_mode : Outport  Port=2
  takeoff_mode : Outport  Port=3
  pos_mode_alt : Outport  Port=4
  master_alt_mode : Outport  Port=5
  sbus_init&ESC1 : Outport  Port=6
  tag scope: CH5_BOOL=global
  wires:
  Logical Operator4/1 -> Logical Operator/1, return_mode/1
  Logical Operator/1 -> Logical Operator6/4, Logical Operator2/3, Logical Operator1/1
  sbus_return/1 -> Compare To Constant/1
  Compare To Constant1/1 -> Logical Operator8/2
  Logical Operator1/1 -> pos_mode/1, Logical Operator11/1
  Compare To Constant2/1 -> Logical Operator5/1
  Logical Operator2/1 -> Logical Operator10/1, takeoff_mode/1
  sbus_alt/1 -> Compare To Constant3/1
  Compare To Constant3/1 -> master_alt_mode/1, Logical Operator3/1
  Compare To Constant/1 -> Logical Operator7/2
  PosCtlSwitch/1 -> Logical Operator4/2, Logical Operator1/3, Logical Operator2/4, Logical Operator6/5
  sbus_init&ESC/1 -> Compare To Constant4/1
  Compare To Constant4/1 -> [CH5_BOOL], PosCtlSwitch/2, sbus_init&ESC1/1
  Compare To Constant5/1 -> Logical Operator6/2
  sbus_pos/1 -> Compare To Constant5/1, Compare To Constant6/1, Compare To Constant2/1, Compare To Constant1/1
  Compare To Constant6/1 -> Logical Operator5/2
  Logical Operator5/1 -> Logical Operator9/2
  Logical Operator6/1 -> pos_mode_alt/1
  return_flag/1 -> Compare To Constant7/1
  Compare To Constant7/1 -> Logical Operator7/1
  Logical Operator7/1 -> Logical Operator4/1
  pos_flag/1 -> Compare To Constant8/1
  Compare To Constant8/1 -> Logical Operator8/1
  Logical Operator8/1 -> Logical Operator1/2
  take_off_flag/1 -> Compare To Constant9/1
  Logical Operator9/1 -> Logical Operator2/2
  Compare To Constant9/1 -> Logical Operator9/1
  Logical Operator10/1 -> Logical Operator6/1
  Logical Operator11/1 -> Logical Operator6/3, Logical Operator2/1
  Logical Operator3/1 -> PosCtlSwitch/1

== system ZF02HD250606_23a/SensorModel/BattV ==
  V3V : Inport
  Add : Sum
  Constant : Constant  Value=-0.2372
  Gain : Gain  Gain=10.7652
  Batt_V : Outport
  wires:
  V3V/1 -> Gain/1
  Gain/1 -> Add/1
  Add/1 -> Batt_V/1  "Batt_V"
  Constant/1 -> Add/2

== system ZF02HD250606_23a/SensorModel/Subsystem ==
  mx : Inport
  my : Inport  Port=2
  Add : Sum
  Add1 : Sum
  Atan2 : Trigonometry  Operator=atan2
  Constant : Constant  Value=1.01
  Constant1 : Constant  Value=-1.09
  Gain : Gain  Gain=-1
  Radians to Degrees : simulink_extras/Transformations/Radians to Degrees
  angle : Outport
  wires:
  my/1 -> Add/1
  mx/1 -> Add1/1
  Add/1 -> Atan2/1
  Add1/1 -> Atan2/2
  Radians to Degrees/1 -> Gain/1
  Gain/1 -> angle/1
  Atan2/1 -> Radians to Degrees/1
  Constant/1 -> Add/2
  Constant1/1 -> Add1/2

== system ZF02HD250606_23a/BasicModel/AttiAltHold/ReturnShutOff ==
  Throttle : Inport
  H /cm : Inport  Port=2
  Compare To Constant1 : simulink/Logic and Bit Operations/Compare To Constant  relop=<=  const=270  OutDataTypeStr=boolean
  Logical Operator1 : Logic  AllPortsSameDT=off  OutDataTypeStr=boolean
  Logical Operator2 : Logic  AllPortsSameDT=off  OutDataTypeStr=boolean
  Logical Operator3 : Logic  Operator=NOT  AllPortsSameDT=off  OutDataTypeStr=boolean
  MATLAB Function : MATLAB Function  TreatAsAtomicUnit=on
  Memory : Memory
  Subsystem : Subsystem  mask{iValue=0.1}
      mask prompts: iValue "请输入每步递减量："
      mask DialogControl ParameterGroupVar Prompt: 每步自减量录入
  Switch : Switch  Criteria=u2 > Threshold  SaturateOnIntegerOverflow=off  InputSameDT=off
  iThrottle : Outport
  FlySts : Outport  Port=2
  wires:
  Switch/1 -> Compare To Constant1/1, Memory/1, iThrottle/1
  Throttle/1 -> Switch/3
  H /cm/1 -> MATLAB Function/2(height)
  MATLAB Function/1(flag) -> Logical Operator1/2, Switch/2
  [return_mode] -> MATLAB Function/1(returnFlg)
  Subsystem/1(Out1) -> Switch/1
  Memory/1 -> Subsystem/1(In1)
  Compare To Constant1/1 -> Logical Operator1/1
  Logical Operator2/1 -> FlySts/1
  Logical Operator1/1 -> Logical Operator3/1  "shuttOff"
  [sbus_init_ESC] -> Logical Operator2/2
  Logical Operator3/1 -> Logical Operator2/1

== system ZF02HD250606_23a/BasicModel/AttiAltHold/Subsystem ==
  VelZ : Inport
  Throttle : Inport  Port=2
  RollDeg : Inport  Port=3
  PitchDeg : Inport  Port=4
  Abs : Abs  SaturateOnIntegerOverflow=off
  Abs1 : Abs  SaturateOnIntegerOverflow=off
  Abs2 : Abs  SaturateOnIntegerOverflow=off
  Compare To Constant1 : simulink/Logic and Bit Operations/Compare To Constant  relop=<  const=60  OutDataTypeStr=boolean
  Compare To Constant2 : simulink/Logic and Bit Operations/Compare To Constant  relop=<  const=500  OutDataTypeStr=boolean
  Compare To Constant3 : simulink/Logic and Bit Operations/Compare To Constant  relop=>  const=190  OutDataTypeStr=boolean
  Compare To Constant4 : simulink/Logic and Bit Operations/Compare To Constant  relop=<  const=500  OutDataTypeStr=boolean
  If : If  IfExpression=u1 ~= 0
  If Action Subsystem : Subsystem  TreatAsAtomicUnit=on
  If Action Subsystem1 : Subsystem  TreatAsAtomicUnit=on
  Memory : Memory
  Merge : Merge
  PosCtlSwitch : Logic  Inputs=4  AllPortsSameDT=off  OutDataTypeStr=boolean
  ThroHove : Outport
  wires:
  Abs2/1 -> Compare To Constant4/1
  PosCtlSwitch/1 -> If/1
  Compare To Constant3/1 -> PosCtlSwitch/1
  RollDeg/1 -> Abs1/1
  PitchDeg/1 -> Abs2/1
  If/2 -> If Action Subsystem1/Action
  If Action Subsystem/1(ThrottHover) -> Merge/1
  Abs/1 -> Compare To Constant1/1
  Memory/1 -> ThroHove/1, If Action Subsystem1/1(In1), If Action Subsystem/2(preThrottHover)  "HoverThrottle"
  Compare To Constant2/1 -> PosCtlSwitch/3
  Abs1/1 -> Compare To Constant2/1
  Compare To Constant4/1 -> PosCtlSwitch/4
  Compare To Constant1/1 -> PosCtlSwitch/2
  If/1 -> If Action Subsystem/Action
  Merge/1 -> Memory/1
  If Action Subsystem1/1(Out1) -> Merge/2
  Throttle/1 -> If Action Subsystem/1(iThrottle), Compare To Constant3/1
  VelZ/1 -> Abs/1

== system ZF02HD250606_23a/BasicModel/AttiAltHold/h_fusion1 ==
  H : Inport
  gps_pos_z : Inport  Port=2
  Vz : Inport  Port=3
  v_neg : Inport  Port=4
  starN : Inport  Port=5
  Add : Sum  Inputs=+-
  Add1 : Sum
  Constant : Constant
  Constant1 : Constant  Value=35
  Gain : Gain  Gain=1/35
  Gain2 : Gain  Gain=-1
  MATLAB Function : MATLAB Function  TreatAsAtomicUnit=on
  Product : Product
  Product1 : Product
  Switch : Switch  Criteria=u2 > Threshold  SaturateOnIntegerOverflow=off  InputSameDT=off
  Switch1 : Switch  Criteria=u2 > Threshold  Threshold=35  SaturateOnIntegerOverflow=off  InputSameDT=off
  judgement : Subsystem
  H_fusion : Outport
  Vz_fusion : Outport  Port=2
  wires:
  H/1 -> MATLAB Function/2(H)
  gps_pos_z/1 -> MATLAB Function/3(gps_NEG_h)
  [nanod_sts] -> MATLAB Function/1(nonod_sts)
  MATLAB Function/1(fusedHeight) -> H_fusion/1
  Add1/1 -> Switch/1
  Switch1/1 -> Gain/1
  judgement/1(flag) -> Switch/2
  Add/1 -> Product1/1
  Constant/1 -> Add/1
  Vz/1 -> Product1/2, Switch/3
  Gain2/1 -> Product/1
  Product/1 -> Add1/1
  Constant1/1 -> Switch1/1
  starN/1 -> judgement/1(starN), Switch1/3, Switch1/2
  Switch/1 -> Vz_fusion/1
  Gain/1 -> Product/2, Add/2
  v_neg/1 -> Gain2/1
  Product1/1 -> Add1/2

== system ZF02HD250606_23a/BasicModel/Tx02/Subsystem2 ==
  lat_in : Inport
  lon_in : Inport  Port=2
  Add : Sum  Inputs=+-
  Add1 : Sum  Inputs=+-
  Constant : Constant  Value=22.801
  Constant1 : Constant  Value=113.948
  Gain : Gain  Gain=100000
  Gain1 : Gain  Gain=100000
  lat_out : Outport
  lon_out : Outport  Port=2
  wires:
  Add1/1 -> Gain1/1
  Gain1/1 -> lon_out/1
  lon_in/1 -> Add1/1
  Constant1/1 -> Add1/2
  Constant/1 -> Add/2
  lat_in/1 -> Add/1
  Gain/1 -> lat_out/1
  Add/1 -> Gain/1

== system ZF02HD250606_23a/NavigationModel/ Navigation Control （X,Y,Z）/POS_CONTROL ==
  note: 位置PI控制
  XYZ_cmd : Inport
  XYZ_bak : Inport  Port=2
  ClrKi : Inport  Port=3
  Add1 : Sum  Inputs=+-
  Demux : Demux  Outputs=3
  Discrete-Time Integrator : DiscreteIntegrator  ExternalReset=level  SampleTime=-1  LimitOutput=on  UpperSaturationLimit=0.6  LowerSaturationLimit=-0.6  ICPrevOutput=DiscIntNeverNeededParam  ICPrevScaledInput=DiscIntNeverNeededParam
  Mux : Mux  Inputs=3
  POS_KI : Gain  Gain=[0.01 0.01 0.02]
  POS_KP1 : Gain  Gain=[0.7 0.7 0.4]
  Reshape : Reshape
  Saturation2 : Saturate  UpperLimit=3  LowerLimit=-3
  Saturation3 : Saturate  UpperLimit=3  LowerLimit=-3
  Saturation4 : Saturate  UpperLimit=1  LowerLimit=-1
  Subtract5 : Sum
  Vxyz_cmd : Outport
  wires:
  Add1/1 -> Reshape/1
  XYZ_bak/1 -> Add1/2
  XYZ_cmd/1 -> Add1/1  "XYZ_cmd"
  POS_KP1/1 -> Subtract5/1
  Mux/1 -> Vxyz_cmd/1
  Demux/1 -> Saturation2/1
  Demux/2 -> Saturation3/1
  Demux/3 -> Saturation4/1
  Saturation2/1 -> Mux/1
  Saturation3/1 -> Mux/2
  Saturation4/1 -> Mux/3
  Reshape/1 -> POS_KP1/1, POS_KI/1
  ClrKi/1 -> Discrete-Time Integrator/2
  Subtract5/1 -> Demux/1
  Discrete-Time Integrator/1 -> Subtract5/2
  POS_KI/1 -> Discrete-Time Integrator/1

== system ZF02HD250606_23a/NavigationModel/ Navigation Control （X,Y,Z）/SETPOINT ==
  posxy : Inport
  pos_mode : Inport  Port=2
  return_mode : Inport  Port=3
  takeoff_mode : Inport  Port=4
  xyz_cmd : Inport  Port=5
  FLAG : Inport  Port=6
  XYZ_bak : Inport  Port=7
  Merge : Merge  Inputs=3
  Merge1 : Merge  Inputs=3
  Mux : Mux  Inputs=2
  Selector : Selector  InputPortWidth=3  IndexOptions=Index vector (dialog)  Indices=[1 2]  OutputSizes=1
  Selector1 : Selector  InputPortWidth=3  IndexOptions=Index vector (dialog)  Indices=3  OutputSizes=1
  Subsystem : Subsystem
  return_mode1 : Subsystem  mask{landing_pos=[0 0 0], decision_h=6, accept_radius=0.4, accept_radius_h=0.5}
      mask DialogControl ParameterGroupVar Prompt: 参数
  setpoints1 : Subsystem  mask{setpoints=[10 0 -4;10 10 -4;0 10 -4;0 0 -4], accept_radius_1=0.4}
      mask DialogControl ParameterGroupVar Prompt: 参数
  takeoff2 : Subsystem  mask{setpoint1=[0 0], takeoff_h=-4}
      mask DialogControl ParameterGroupVar Prompt: 参数
  XYZ_cmd : Outport
  Flag : Outport  Port=2
  wires:
  posxy/1 -> return_mode1/2(posxy)
  return_mode1/1(setpoint_next) -> Merge/3  "XYZ_cmd"
  Mux/1 -> return_mode1/1(pos1), setpoints1/1(pos1)  "XYZ"
  setpoints1/1(setpoint_next) -> Merge/2  "XYZ_cmd"
  return_mode/1 -> return_mode1/Enable
  pos_mode/1 -> setpoints1/Enable
  Selector/1 -> Subsystem/2(pos), Mux/1  "XY"
  Selector1/1 -> takeoff2/2(h), Mux/2
  takeoff_mode/1 -> takeoff2/Enable, Subsystem/1(takeoff)
  takeoff2/1(setpoint_next) -> Merge/1  "XYZ_cmd"
  xyz_cmd/1 -> setpoints1/2(xyz_cmd)
  FLAG/1 -> setpoints1/3(FLAG)
  Subsystem/1(posxy) -> takeoff2/1(posxy)
  Merge/1 -> XYZ_cmd/1
  Merge1/1 -> Flag/1
  setpoints1/2(Flag) -> Merge1/2
  takeoff2/2(flag) -> Merge1/1
  return_mode1/2(flag) -> Merge1/3
  XYZ_bak/1 -> Selector1/1, Selector/1
